simulink model "afe_inv_psm_param"  (R2026b)
settings: Solver=ode23t  StopTime=param.sim.simlength  FixedStep=tc  MaxStep=param.glb_time.tc  RelTol=1e-4
values from neighbouring files (symbols this model uses):
  param = add_template_extras(param, options)    [init_model.m]
undefined symbols (not defined in the file or in its folder): magnitude, omega_m_bez
libraries: fl_lib x330, nesl_utility x174, igbt_simple_2th_lib x12, moving_average_filter x10, moving_average_filter_cc x8, sl_discontinuities x3, single_phase_transformer_lib x3, linear_double_integrator_observer_ccaller x2, discrete_time_low_pass_filter x2, threephase_inductor_lib x2, three_phase_pwm_modulator x2, three_phase_inverter_ideal_switch_based_model x2
(part 13 of 13)

== system afe_inv_psm_param/afe_abc_inv_psm_mod1/INV_control/inverter_control/current_ctrl/current_ctrl/dq_pi_with_vector_antiwindup mod1/dq_vector_pi/vector lenght ==
  md : Inport
  mq : Inport  Port=2
  Math Function : Math  Operator=magnitude^2  SignedPower=on
  Math Function1 : Math  Operator=magnitude^2  SignedPower=on
  Math Function2 : Math  Operator=reciprocal  SignedPower=on
  Sqrt : Sqrt
  Sum5 : Sum  SaturateOnIntegerOverflow=on
  m_1 : Outport  VectorParamsAs1DForOutWhenUnconnected=off
  m : Outport  Port=2  VectorParamsAs1DForOutWhenUnconnected=off
  wires:
  Sqrt/1 -> m/1, Math Function2/1
  mq/1 -> Math Function1/1
  Math Function1/1 -> Sum5/2
  Math Function/1 -> Sum5/1
  Sum5/1 -> Sqrt/1
  Math Function2/1 -> m_1/1
  md/1 -> Math Function/1

== system afe_inv_psm_param/afe_abc_inv_psm_mod1/INV_control/inverter_control/current_ctrl/current_ctrl/dq_pi_with_vector_antiwindup mod1/dq_vector_pi_ccaller/Reset ==
  Step : Step  Time=0.05  InitialValue=1  FinalValue=0
  en : Outport
  wires:
  Step/1 -> en/1

== system afe_inv_psm_param/afe_abc_inv_psm_mod1/INV_control/inverter_control/current_ctrl/bemf_observer/EKF_bemf_observer/extended_kalman_observer/correlation_matrix/A_ekf ==
  Gain1 : Gain  Gain=param.psm.ctrl.ekf.A6_tilde_ekf
  Gain{7..10,13,20} (6 alike) : Gain  Gain=param.psm.machine.omega_bez
  Gain{2,4,6,11,16,18} (6 alike) : Gain  Gain=param.glb_time.ts_inv
  Gain15 : Gain  Gain=param.psm.ctrl.ekf.A2_tilde_ekf
  Gain17 : Gain  Gain=param.psm.ctrl.ekf.A3_tilde_ekf
  Gain3 : Gain  Gain=param.psm.ctrl.ekf.A4_tilde_ekf
  Gain5 : Gain  Gain=param.psm.ctrl.ekf.A5_tilde_ekf
  I1 : Constant  Value=eye(6)
  I2 : Constant  Value=param.psm.ctrl.ekf.A1_tilde_ekf
  Sum7 : Sum  Inputs=+++++++
  out : Outport
  wires:
  Sum7/1 -> out/1
  I2/1 -> Gain11/1
  I1/1 -> Sum7/1
  Gain1/1 -> Gain2/1
  Gain3/1 -> Gain4/1
  Gain5/1 -> Gain6/1
  [omega_hat_kalman] -> Gain1/1
  [psi_alpha_hat] -> Gain3/1
  [psi_beta_hat] -> Gain5/1
  Gain11/1 -> Gain7/1
  Gain2/1 -> Gain8/1
  Gain4/1 -> Gain9/1
  Gain6/1 -> Gain10/1
  Gain7/1 -> Sum7/2
  Gain9/1 -> Sum7/5
  Gain10/1 -> Sum7/6
  Gain8/1 -> Sum7/7
  Gain18/1 -> Gain13/1
  Gain16/1 -> Gain20/1
  Gain17/1 -> Gain18/1
  Gain15/1 -> Gain16/1
  Gain13/1 -> Sum7/4
  Gain20/1 -> Sum7/3
  [i_beta_hat] -> Gain17/1
  [i_alpha_hat] -> Gain15/1

== matlab function afe_inv_psm_param/afe_abc_inv_psm_mod1/AFE_control/afe_control/current_ctrl/current_transformation/alphabeta2xieta ==
  data: alpha input; xi output; beta input; gamma input; eta output
function [xi,eta] = alphabeta2xieta(alpha,beta,gamma)

    xi  =  alpha*cos(gamma) + beta*sin(gamma);
    eta = -alpha*sin(gamma) + beta*cos(gamma);

end

== matlab function afe_inv_psm_param/afe_abc_inv_psm_mod1/AFE_control/afe_control/grid_voltage_phase_lock_loops/FHT-PLL/pll_stageB/bounder1 ==
  data: u input; y output
function y = bounder(u)
    y = -pi + mod(u+3*pi,2*pi);
end

== matlab function afe_inv_psm_param/afe_abc_inv_psm_mod1/INV_control/inverter_control/current_ctrl/current_transformation/uvw2alphabeta ==
  data: u input; alpha output; v input; w input; beta output
function [alpha,beta] = uvw2alphabeta(u,v,w)

alpha = 2/3*(u - 1/2*v - 1/2*w);
beta  = 2/3*(sqrt(3)/2*(v - w));

end

== matlab function afe_inv_psm_param/afe_abc_inv_psm_mod1/INV_control/inverter_control/current_ctrl/current_ctrl/output voltage transformation/dq2alphabeta ==
  data: d input; alpha output; q input; gamma input; beta output
function [alpha,beta] = dq2alphabeta(d,q,gamma)

    alpha  =  d*cos(gamma) - q*sin(gamma);
    beta = d*sin(gamma) + q*cos(gamma);

end

== matlab function afe_inv_psm_param/afe_abc_inv_psm_mod1/AFE_control/afe_control/FRT-VDE4110/FRT-Detection/LVRT_detector ==
  data: vxi_p input; vxi_n input; veta_n input; vxi_p_dot input; vxi_n_dot input; enable input; red_dyn_enabled input; pwr_lim_enable output; frt_exceeded output; reset input; frt_active output; frt_state output; red_dyn_active output
function [pwr_lim_enable, frt_exceeded, frt_active, frt_state, red_dyn_active]  = lvrt_detector(vxi_p,vxi_n,veta_n,vxi_p_dot,vxi_n_dot, enable, red_dyn_enabled, reset)

    persistent state count count2 state_pwr_lim
    
    LVRT_IDLE = 0;
    LVRT_ACTIVE = 1;
    LVRT_EXCEEDED = 2;
    
    PWR_LIM_DISABLED = 0;
    PWR_LIM_ENABLED  = 1;
    
    LVRT_VPOS_TH_LOW			= 0.85;
    LVRT_VPOS_TH_HIGH			= 1.15;
    LVRT_SEQ_DETECTION_HYST		= 0.1;
    LVRT_VNEG_TH				= 0.1;
    LVRT_VPOS_DOT_TH			= 2.0;
    LVRT_VNEG_DOT_TH			= 2.0;
    LVRT_VPOS_PWRLIM_TH			= 0.8;
    LVRT_VNEG_PWRLIM_TH			= 0.1;
    LVRT_PWRLIM_HYST			= 0.1;
    LVRT_VPOS_RED_DYN_TH        = 0.7;
    LVRT_VNEG_RED_DYN_TH        = 0.2;
    LVRT_TIME_HOLD_MAX          = 61000;
    
    RED_DYN_NOT_ACTIVE = 0;
    RED_DYN_ACTIVE     = 1;
        
    if isempty(state)
        state = LVRT_IDLE;
        state_pwr_lim = PWR_LIM_DISABLED;
        count = 0;
        count2 = 0;
    end

    vn = sqrt(vxi_n^2+veta_n^2);

    if enable == 1
        
        switch state
            
            case LVRT_IDLE
                if ((vxi_p > LVRT_VPOS_TH_HIGH || vxi_p < LVRT_VPOS_TH_LOW || vn > LVRT_VNEG_TH) ...
                     && (vxi_p_dot > LVRT_VPOS_DOT_TH || vxi_n_dot > LVRT_VNEG_DOT_TH) && ...
                     count2 > 1000)
                    state = LVRT_ACTIVE;
                end
                frt_active = 0;
                frt_exceeded = 0;
                count = 0;
                frt_state = LVRT_IDLE;
                state_pwr_lim = PWR_LIM_DISABLED;                  
                red_dyn_active = RED_DYN_NOT_ACTIVE;
                count2 = count2 + 1;

            case LVRT_ACTIVE
                count2 = 0;
                % LVRT condition not active anymore
                if (vxi_p >= LVRT_VPOS_TH_LOW  + LVRT_SEQ_DETECTION_HYST && ...
                    vxi_p <  LVRT_VPOS_TH_HIGH - LVRT_SEQ_DETECTION_HYST)
                    state = LVRT_IDLE;
                % LVRT exceeded
                elseif (count >= LVRT_TIME_HOLD_MAX)
                    state = LVRT_EXCEEDED;
                end
                
                % handle power limitation
                if (vxi_p < LVRT_VPOS_PWRLIM_TH || vn > LVRT_VNEG_PWRLIM_TH) 
                    state_pwr_lim = PWR_LIM_ENABLED;
                elseif (vxi_p > LVRT_VPOS_PWRLIM_TH + LVRT_PWRLIM_HYST && vn < LVRT_VPOS_PWRLIM_TH - LVRT_PWRLIM_HYST)
                    state_pwr_lim = PWR_LIM_DISABLED;                  
                end
                
                % handle reduced dynamic grid support
                if red_dyn_enabled && (vxi_p < LVRT_VPOS_RED_DYN_TH || vn > LVRT_VNEG_RED_DYN_TH)
                    red_dyn_active = RED_DYN_ACTIVE;
                else
                    red_dyn_active = RED_DYN_NOT_ACTIVE;
                end
                 
                frt_active = 1;
                frt_exceeded = 0;
                frt_state = LVRT_ACTIVE;
                
                count = count + 1;
            
            case LVRT_EXCEEDED

                if ((reset == 1) || (enable == 0))
                    state = LVRT_IDLE;
                else
                    state = LVRT_EXCEEDED;
                end
                
                frt_exceeded = 1;
                frt_active = 0; 
                frt_state = LVRT_EXCEEDED;
                red_dyn_active = RED_DYN_NOT_ACTIVE;
            
            otherwise
                state = LVRT_IDLE;
                frt_active = 0;
                frt_exceeded = 0;
                frt_state = LVRT_IDLE;
                red_dyn_active = RED_DYN_NOT_ACTIVE;
        end
        
        if state_pwr_lim == PWR_LIM_ENABLED
            pwr_lim_enable = 1;
        else
            pwr_lim_enable = 0;
        end      
    else
        state = LVRT_IDLE;
        frt_active = 0;
        pwr_lim_enable = 0;
        frt_exceeded = 0;
        frt_state = LVRT_IDLE;
        red_dyn_active = RED_DYN_NOT_ACTIVE;
    end
end

== matlab function afe_inv_psm_param/afe_abc_inv_psm_mod1/brake/MATLAB Function ==
  data: u input; y output; udc_ref input
function y = fcn(u,udc_ref)

persistent enable_brake

udc_brake_min = 1.15;
udc_brake_max = 1.175;

if isempty(enable_brake)
    enable_brake = 0
end

if u >= udc_ref*udc_brake_max
    y = 15;
    enable_brake = 1;
elseif (u < udc_ref*udc_brake_max && u >= udc_ref*udc_brake_min && enable_brake == 1)
    y = 15;
    enable_brake = 1;
elseif (u < udc_ref*udc_brake_max && u >= udc_ref*udc_brake_min && enable_brake == 0)
    y = 0;
    enable_brake = 0;
else
    y = 0;
    enable_brake = 0;
end

% function y = fcn(u,udc_ref)
% 
% persistent enable_brake
% 
% udc_brake_min = 1.145;
% udc_brake_max = 1.165;
% 
% if isempty(enable_brake)
%     enable_brake = 0
% end
% 
% if u >= udc_ref*udc_brake_max
%     y = 15;
%     enable_brake = 1;
% elseif (u < udc_ref*udc_brake_max && u >= udc_ref*udc_brake_min && enable_brake == 1)
%     y = 15;
%     enable_brake = 1;
% elseif (u < udc_ref*udc_brake_max && u >= udc_ref*udc_brake_min && enable_brake == 0)
%     y = 0;
%     enable_brake = 0;
% else
%     y = 0;
%     enable_brake = 0;
end

== matlab function afe_inv_psm_param/afe_abc_inv_psm_mod1/AFE_control/afe_control/grid_voltage_phase_lock_loops/FHT-PLL/pll_stageB/double_integrator_observer/bounder1 ==
  data: u input; y output
function y = bounder(u)
    
    y = -pi + mod(u+3*pi,2*pi);
    
end

== matlab function afe_inv_psm_param/afe_abc_inv_psm_mod1/AFE_control/afe_control/grid_voltage_phase_lock_loops/FHT-PLL/pll_stageB/double_integrator_observer/bounder2 ==
  data: u input; y output
function y = bounder(u)
    
    y = -pi + mod(u+3*pi,2*pi);
    
end

== matlab function afe_inv_psm_param/afe_abc_inv_psm_mod1/INV_control/inverter_control/current_ctrl/bemf_observer/EKF_bemf_observer/extended_kalman_observer/double_integrator_observer/bounder2 ==
  data: u input; y output
function y = bounder(u)
    y = -pi + mod(u+3*pi,2*pi);
end

== matlab function afe_inv_psm_param/afe_abc_inv_psm_mod1/AFE_control/afe_control/grid_voltage_phase_lock_loops/FHT-PLL_simulink/pll_stageA/filter_and_transformation/abc2alphabeta ==
  data: a input; alpha output; b input; c input; beta output
function [alpha,beta] = abc2alphabeta(a,b,c)

alpha = 2/3*(a - 1/2*b - 1/2*c);
beta  = 1/sqrt(3)*(b - c);

end

== matlab function afe_inv_psm_param/afe_abc_inv_psm_mod1/AFE_control/afe_control/grid_voltage_phase_lock_loops/FHT-PLL_simulink/pll_stageA/sequences/alphabeta2xieta ==
  data: alpha input; xi output; beta input; gamma input; eta output
function [xi,eta] = alphabeta2xieta_pos(alpha,beta,gamma)

    xi  =  (alpha*cos(gamma) + beta*sin(gamma));
    eta = (-alpha*sin(gamma) + beta*cos(gamma));

end

== matlab function afe_inv_psm_param/afe_abc_inv_psm_mod1/AFE_control/afe_control/grid_voltage_phase_lock_loops/FHT-PLL_simulink/pll_stageB/bounder1 ==
  data: u input; y output
function y = bounder(u)
    y = -pi + mod(u+3*pi,2*pi);
end

== matlab function afe_inv_psm_param/afe_abc_inv_psm_mod1/AFE_control/afe_control/grid_voltage_phase_lock_loops/FHT-PLL_simulink/pll_stageB/double_integrator_observer/bounder1 ==
  data: u input; y output
function y = bounder(u)
    
    y = -pi + mod(u+3*pi,2*pi);
    
end

== matlab function afe_inv_psm_param/afe_abc_inv_psm_mod1/AFE_control/afe_control/grid_voltage_phase_lock_loops/dq_pll/pll_stageA/mormalization_and_transformation/abc2alphabeta ==
  data: a input; alpha output; b input; c input; beta output
function [alpha,beta] = abc2alphabeta(a,b,c)

alpha = 2/3*(a - 1/2*b - 1/2*c);
beta  = 1/sqrt(3)*(b - c);

end

== matlab function afe_inv_psm_param/afe_abc_inv_psm_mod1/AFE_control/afe_control/grid_voltage_phase_lock_loops/dq_pll/pll_stageA/sequences/alphabeta2xieta/alphabeta2xieta_neg ==
  data: alpha input; xi output; beta input; gamma input; eta output
function [xi,eta] = alphabeta2xieta_neg(alpha,beta,gamma)

    xi  = alpha*cos(gamma) - beta*sin(gamma);
    eta = alpha*sin(gamma) + beta*cos(gamma);

end

== matlab function afe_inv_psm_param/afe_abc_inv_psm_mod1/AFE_control/afe_control/grid_voltage_phase_lock_loops/dq_pll/pll_stageA/sequences/alphabeta2xieta/alphabeta2xieta_pos ==
  data: alpha input; xi output; beta input; gamma input; eta output
function [xi,eta] = alphabeta2xieta_pos(alpha,beta,gamma)

    xi  =  alpha*cos(gamma) + beta*sin(gamma);
    eta = -alpha*sin(gamma) + beta*cos(gamma);

end

== matlab function afe_inv_psm_param/afe_abc_inv_psm_mod1/INV_control/inverter_control/current_ctrl/bemf_observer/bemf_observer/double_integrator_observer/bounder1 ==
  data: u input; y output
function y = bounder(u)
    
    y = -pi + mod(u+3*pi,2*pi);
end

== matlab function afe_inv_psm_param/afe_abc_inv_psm_mod1/INV_control/inverter_control/current_ctrl/bemf_observer/bemf_observer/double_integrator_observer/bounder2 ==
  data: u input; y output
function y = bounder(u)
    
    u = -pi + mod(u+3*pi,2*pi);
    
    y = u;
end

== matlab function afe_inv_psm_param/afe_abc_inv_psm_mod1/AFE_control/afe_control/FRT-VDE4110/FRT-PosNegReactiveCurrentReferences/avg_flt_500ms/avg_flt_1 ==
  data: x input; y1 output; w input; ts input; enable input
function y1  = avg_flt(x,w,ts, enable)

    persistent x_int x_int_1 y_N N

    N = (1/(w/(2*pi)))/ts+1;

    if isempty(x_int)
        x_int_1 = 0;
        y_N = zeros(1,N);
        y1 = 0;
    end


    if enable == 1
        x_int = x * ts * w + x_int_1;
        x_int_1 = x_int;
        y_N(1,1) = x_int;
        y1 = 1/(2*pi)*((y_N(1,1) - y_N(1,N)));
        for i = 1:(N-1)
            y_N(1,N+1-i) = y_N(1,N-i); 
        end
    else
        y1 = 1/(2*pi)*((y_N(1,1) - y_N(1,N)));
    end
end

== matlab function afe_inv_psm_param/afe_abc_inv_psm_mod1/AFE_control/afe_control/grid_voltage_phase_lock_loops/dq_pll/pll_stageB/double_integrator_observer/bounder1 ==
  data: u input; y output
function y = bounder(u)
    
    y = -pi + mod(u+3*pi,2*pi);
    
end

== matlab function afe_inv_psm_param/afe_abc_inv_psm_mod1/AFE_control/afe_control/islanding_mode_detector/MATLAB Function ==
  data: alpha input; xi output; beta input; gamma input; eta output
function [xi,eta] = alphabeta2pos(alpha,beta,gamma)

    xi  =  alpha*cos(gamma) + beta*sin(gamma);
    eta = -alpha*sin(gamma) + beta*cos(gamma);

end

== matlab function afe_inv_psm_param/afe_abc_inv_psm_mod1/AFE_control/afe_control/grid_voltage_phase_lock_loops/dq_pll/pll_stageB/double_integrator_observer/bounder2 ==
  data: u input; y output
function y = bounder(u)
    
    y = -pi + mod(u+3*pi,2*pi);
    
end

== matlab function afe_inv_psm_param/afe_abc_inv_psm_mod1/AFE_control/afe_control/islanding_mode_detector/bounder ==
  data: u input; y output
function y = bounder(u)
    
    u = -pi + mod(u+3*pi,2*pi);
    
    y = u;
end

== matlab function afe_inv_psm_param/grid/power meter iec mfunc/three_phase_power_meter_iec ==
  data: phase input; m output Bus: PowerMeterIecBus; u_abc input; i_abc input; omega input; ts input; enable_time input
function m = three_phase_power_meter_iec(phase, u_abc, i_abc, omega, ts, enable_time)
%#codegen
% THREE_PHASE_POWER_METER_IEC
% Equivalente in singolo blocco MATLAB Function del sottosistema Simulink
% "three_phase_power_meter_iec" (libreria power_meter_iec).
%
% INGRESSI
%   phase       : angolo del PLL [rad]      (scalare)
%   u_abc       : tensioni di fase [V]      (3x1)
%   i_abc       : correnti di linea [A]     (3x1)
%   omega       : pulsazione di rete [rad/s] (scalare)
%   ts          : passo di campionamento [s]  -> parametro di maschera
%   enable_time : istante di abilitazione [s] -> parametro di maschera
%
% USCITA
%   m : struct (bus) con i campi, nello stesso ordine del Bus Creator
%       originale: Q1p, Q1n, P1n, P1p, U1n, U1p,
%                  i_act_1n, i_react_1n, i_act_1p, i_react_1p
%
% CATENA DI ELABORAZIONE (identica all'originale)
%   1) proiezione di ogni fase su cos(phase) e sin(phase), guadagno 2
%   2) media mobile dinamica su finestra pari a mezzo periodo di rete
%      (Tw = pi/|omega|), con lunghezza frazionaria interpolata
%   3) componenti simmetriche di sequenza diretta e inversa (Fortescue)
%   4) potenze attiva e reattiva per sequenza, tensioni concatenate RMS,
%      correnti attiva e reattiva per sequenza
%
% NOTE
%   - Il blocco deve girare a passo fisso ts (gli Zero-Order Hold di
%     ingresso dell'originale sono impliciti nel sample time del blocco).
%   - ts ed enable_time possono essere dichiarati come dati di scope
%     "Parameter" nel Symbols pane del MATLAB Function block, cosi'
%     risolvono direttamente sui parametri di maschera e la firma
%     esterna resta a 4 ingressi come nel blocco originale.

% ------------------------------------------------------------------
% Costanti
% ------------------------------------------------------------------
% MAVGFLT_SIZE_MAX = 17500;   % lunghezza buffer circolare (come originale)
MAVGFLT_SIZE_MAX = 2048;   % lunghezza buffer ridotto
NCH              = 12;      % canali filtrati: 6 per u_abc, 6 per i_abc

% Ordine canali:
%   1..3  ua_cos ub_cos uc_cos      7..9   ia_cos ib_cos ic_cos
%   4..6  ua_sin ub_sin uc_sin     10..12  ia_sin ib_sin ic_sin

% ------------------------------------------------------------------
% Stato persistente
% ------------------------------------------------------------------
persistent buf cb_index sample_count sum_short sum_long prev_input ...
           k_step period_held

if isempty(buf)
    buf          = zeros(NCH, MAVGFLT_SIZE_MAX);
    cb_index     = ones(NCH, 1);
    sample_count = ones(NCH, 1);
    sum_short    = zeros(NCH, 1);
    sum_long     = zeros(NCH, 1);
    prev_input   = zeros(NCH, 1);
    k_step       = 0;
    period_held  = 0;          % uscita iniziale dell'Enabled Subsystem
end

% ------------------------------------------------------------------
% Abilitazione (equivalente al blocco Step con Time = enable_time)
% ------------------------------------------------------------------
t_now  = k_step * ts;
k_step = k_step + 1;
enable = (t_now >= enable_time);

% ------------------------------------------------------------------
% Finestra di media: Enabled Subsystem 2*pi/w, alimentato da 2*|omega|.
% Quando |omega| = 0 l'Enabled Subsystem mantiene l'ultimo valore.
% ------------------------------------------------------------------
w2 = 2 * abs(omega);
if w2 > 0
    period_held = 2*pi / w2;   % = pi/|omega|, mezzo periodo di rete
end
period = period_held;

% ------------------------------------------------------------------
% Proiezione sin/cos, guadagno 2
% ------------------------------------------------------------------
c = cos(phase);
s = sin(phase);

x = zeros(NCH, 1);
x(1)  = 2 * u_abc(1) * c;   x(2)  = 2 * u_abc(2) * c;   x(3)  = 2 * u_abc(3) * c;
x(4)  = 2 * u_abc(1) * s;   x(5)  = 2 * u_abc(2) * s;   x(6)  = 2 * u_abc(3) * s;
x(7)  = 2 * i_abc(1) * c;   x(8)  = 2 * i_abc(2) * c;   x(9)  = 2 * i_abc(3) * c;
x(10) = 2 * i_abc(1) * s;   x(11) = 2 * i_abc(2) * s;   x(12) = 2 * i_abc(3) * s;

% ------------------------------------------------------------------
% Banco di 12 filtri a media mobile dinamica (dmavgflt_process)
% ------------------------------------------------------------------
y = zeros(NCH, 1);

if enable && period > 0

    desired = period / ts;
    if desired > (MAVGFLT_SIZE_MAX - 1)
        desired = MAVGFLT_SIZE_MAX - 1;
    end

    n_samples = floor(desired + 1);          % campioni che coprono il periodo
    frac      = desired + 1 - n_samples;     % parte frazionaria
    if n_samples < 1
        n_samples = 1;
    end

    for ch = 1:NCH

        ci = cb_index(ch);
        sc = sample_count(ch);

        if n_samples > sc
            % finestra in crescita: aggiungi campioni
            sum_short(ch) = sum_short(ch) + prev_input(ch);
            sum_long(ch)  = sum_long(ch)  + x(ch);
            sc = sc + 1;

        elseif n_samples < sc
            % finestra in contrazione: rimuovi i due campioni piu' vecchi
            i1 = mod(ci - 1 - sc,       MAVGFLT_SIZE_MAX) + 1;
            i2 = mod(ci - 1 - (sc - 1), MAVGFLT_SIZE_MAX) + 1;
            old_sum = buf(ch, i1) + buf(ch, i2);

            sum_short(ch) = sum_short(ch) + prev_input(ch) - old_sum;
            sum_long(ch)  = sum_long(ch)  + x(ch)          - old_sum;
            sc = sc - 1;

        else
            % finestra costante
            i1     = mod(ci - 1 - sc, MAVGFLT_SIZE_MAX) + 1;
            oldest = buf(ch, i1);

            sum_short(ch) = sum_short(ch) + prev_input(ch) - oldest;
            sum_long(ch)  = sum_long(ch)  + x(ch)          - oldest;
        end

        % aggiornamento buffer circolare
        buf(ch, ci)      = x(ch);
        cb_index(ch)     = mod(ci, MAVGFLT_SIZE_MAX) + 1;
        prev_input(ch)   = x(ch);
        sample_count(ch) = sc;

        % uscita: interpolazione lineare fra finestra corta e lunga
        if sc > 1
            avg_short = sum_short(ch) / (sc - 1);
        else
            avg_short = 0;
        end
        avg_long = sum_long(ch) / sc;

        y(ch) = avg_short * (1 - frac) + avg_long * frac;
    end
end
% se enable = false oppure period <= 0: y resta 0 e lo stato non evolve
% (comportamento identico all'originale)

ua_cos = y(1);  ub_cos = y(2);  uc_cos = y(3);
ua_sin = y(4);  ub_sin = y(5);  uc_sin = y(6);
ia_cos = y(7);  ib_cos = y(8);  ic_cos = y(9);
ia_sin = y(10); ib_sin = y(11); ic_sin = y(12);

% ------------------------------------------------------------------
% Componenti simmetriche (fasori con convenzione U = u_cos - j*u_sin)
% ------------------------------------------------------------------
sq3 = sqrt(3);

u1p_cos = (2*ua_cos - ub_cos - uc_cos - sq3*(uc_sin - ub_sin)) / 6;
u1p_sin = (2*ua_sin - ub_sin - uc_sin - sq3*(ub_cos - uc_cos)) / 6;
u1n_cos = (2*ua_cos - ub_cos - uc_cos - sq3*(ub_sin - uc_sin)) / 6;
u1n_sin = (2*ua_sin - ub_sin - uc_sin - sq3*(uc_cos - ub_cos)) / 6;

i1p_cos = (2*ia_cos - ib_cos - ic_cos - sq3*(ic_sin - ib_sin)) / 6;
i1p_sin = (2*ia_sin - ib_sin - ic_sin - sq3*(ib_cos - ic_cos)) / 6;
i1n_cos = (2*ia_cos - ib_cos - ic_cos - sq3*(ib_sin - ic_sin)) / 6;
i1n_sin = (2*ia_sin - ib_sin - ic_sin - sq3*(ic_cos - ib_cos)) / 6;

% ------------------------------------------------------------------
% Potenze per sequenza
% ------------------------------------------------------------------
P1p = 1.5 * (u1p_cos*i1p_cos + u1p_sin*i1p_sin);
Q1p = 1.5 * (u1p_cos*i1p_sin - u1p_sin*i1p_cos);
P1n = 1.5 * (u1n_cos*i1n_cos + u1n_sin*i1n_sin);
Q1n = 1.5 * (u1n_cos*i1n_sin - u1n_sin*i1n_cos);

% ------------------------------------------------------------------
% Tensioni concatenate RMS per sequenza: sqrt(3/2)*ampiezza di fase
% ------------------------------------------------------------------
U1p = sqrt(1.5 * (u1p_cos^2 + u1p_sin^2));
U1n = sqrt(1.5 * (u1n_cos^2 + u1n_sin^2));

% ------------------------------------------------------------------
% Correnti attiva e reattiva per sequenza (RMS di linea)
% La protezione contro la divisione per zero non era presente nello
% schema originale (i blocchi Divide restituivano Inf/NaN a U = 0).
% Portare U_MIN a 0 per replicare esattamente il comportamento vecchio.
% ------------------------------------------------------------------
U_MIN = 1e-9;

if U1p > U_MIN
    i_act_1p   = P1p / (sq3 * U1p);
    i_react_1p = Q1p / (sq3 * U1p);
else
    i_act_1p   = 0;
    i_react_1p = 0;
end

if U1n > U_MIN
    i_act_1n   = P1n / (sq3 * U1n);
    i_react_1n = Q1n / (sq3 * U1n);
else
    i_act_1n   = 0;
    i_react_1n = 0;
end

% ------------------------------------------------------------------
% Bus di uscita (stesso ordine dei campi dell'originale)
% ------------------------------------------------------------------
m.Q1p        = Q1p;
m.Q1n        = Q1n;
m.P1n        = P1n;
m.P1p        = P1p;
m.U1n        = U1n;
m.U1p        = U1p;
m.i_act_1n   = i_act_1n;
m.i_react_1n = i_react_1n;
m.i_act_1p   = i_act_1p;
m.i_react_1p = i_react_1p;

end

== matlab function afe_inv_psm_param/afe_abc_inv_psm_mod1/AFE_control/afe_control/current_ctrl/inner_current_ctrl/zero_current_ctrl/antiwind_up/MATLAB Function1 ==
  data: da input; das output; db input; dc input; scaling input; dbs output; dcs output
function [das, dbs, dcs] = fcn(da,db,dc,scaling)

das = da/scaling;
dbs = db/scaling;
dcs = dc/scaling;

== matlab function afe_inv_psm_param/afe_abc_inv_psm_mod1/AFE_control/afe_control/FRT-VDE4110/FRT-PosNegReactiveCurrentReferences/avg_flt_500ms1/avg_flt_1 ==
  data: x input; y1 output; w input; ts input; enable input
function y1  = avg_flt(x,w,ts, enable)

    persistent x_int x_int_1 y_N N

    N = (1/(w/(2*pi)))/ts+1;

    if isempty(x_int)
        x_int_1 = 0;
        y_N = zeros(1,N);
        y1 = 0;
    end


    if enable == 1
        x_int = x * ts * w + x_int_1;
        x_int_1 = x_int;
        y_N(1,1) = x_int;
        y1 = 1/(2*pi)*((y_N(1,1) - y_N(1,N)));
        for i = 1:(N-1)
            y_N(1,N+1-i) = y_N(1,N-i); 
        end
    else
        y1 = 1/(2*pi)*((y_N(1,1) - y_N(1,N)));
    end
end

== matlab function afe_inv_psm_param/afe_abc_inv_psm_mod1/AFE_control/afe_control/FRT-VDE4110/FRT-PosNegReactiveCurrentReferences/avg_flt_500ms2/avg_flt_1 ==
  data: x input; y1 output; w input; ts input; enable input
function y1  = avg_flt(x,w,ts, enable)

    persistent x_int x_int_1 y_N N

    N = (1/(w/(2*pi)))/ts+1;

    if isempty(x_int)
        x_int_1 = 0;
        y_N = zeros(1,N);
        y1 = 0;
    end


    if enable == 1
        x_int = x * ts * w + x_int_1;
        x_int_1 = x_int;
        y_N(1,1) = x_int;
        y1 = 1/(2*pi)*((y_N(1,1) - y_N(1,N)));
        for i = 1:(N-1)
            y_N(1,N+1-i) = y_N(1,N-i); 
        end
    else
        y1 = 1/(2*pi)*((y_N(1,1) - y_N(1,N)));
    end
end

== matlab function afe_inv_psm_param/afe_abc_inv_psm_mod1/AFE_control/afe_control/FRT-VDE4110/FRT-PosNegReactiveCurrentReferences/avg_flt_500ms3/avg_flt_1 ==
  data: x input; y1 output; w input; ts input; enable input
function y1  = avg_flt(x,w,ts, enable)

    persistent x_int x_int_1 y_N N

    N = (1/(w/(2*pi)))/ts+1;

    if isempty(x_int)
        x_int_1 = 0;
        y_N = zeros(1,N);
        y1 = 0;
    end


    if enable == 1
        x_int = x * ts * w + x_int_1;
        x_int_1 = x_int;
        y_N(1,1) = x_int;
        y1 = 1/(2*pi)*((y_N(1,1) - y_N(1,N)));
        for i = 1:(N-1)
            y_N(1,N+1-i) = y_N(1,N-i); 
        end
    else
        y1 = 1/(2*pi)*((y_N(1,1) - y_N(1,N)));
    end
end

== matlab function afe_inv_psm_param/afe_abc_inv_psm_mod1/AFE_control/afe_control/grid_voltage_sequences/v_alphabeta2xieta/MATLAB Function ==
  data: alpha input; xi output; beta input; gamma input; eta output
function [xi,eta] = alphabeta2pos(alpha,beta,gamma)

    xi  =  alpha*cos(gamma) + beta*sin(gamma);
    eta = -alpha*sin(gamma) + beta*cos(gamma);

end

== matlab function afe_inv_psm_param/afe_abc_inv_psm_mod1/AFE_control/afe_control/grid_voltage_sequences/v_alphabeta2xieta/MATLAB Function1 ==
  data: alpha input; xi output; beta input; gamma input; eta output
function [xi,eta] = alphabeta2neg(alpha,beta,gamma)

    xi  = alpha*cos(gamma) - beta*sin(gamma);
    eta = alpha*sin(gamma) + beta*cos(gamma);

end

== matlab function afe_inv_psm_param/afe_abc_inv_psm_mod1/AFE_control/afe_control/grid_voltage_sequences/grid_voltage_sampling_and_alpha_beta_transformation/v_abc2alphabeta ==
  data: v_abc input; alpha output; beta output
function [alpha,beta] = abc2alphabeta(v_abc)

alpha = 2/3*(v_abc(1) - 1/2*v_abc(2) - 1/2*v_abc(3));
beta  = 1/sqrt(3)*(v_abc(2) - v_abc(3));

end

== matlab function afe_inv_psm_param/afe_abc_inv_psm_mod1/AFE_control/afe_control/grid_current_sequences_and_reactive_pwr_ctrl/i_alphabeta2xieta/MATLAB Function ==
  data: alpha input; xi output; beta input; gamma input; eta output
function [xi,eta] = alphabeta2pos(alpha,beta,gamma)

    xi  =  alpha*cos(gamma) + beta*sin(gamma);
    eta = -alpha*sin(gamma) + beta*cos(gamma);

end

== matlab function afe_inv_psm_param/afe_abc_inv_psm_mod1/AFE_control/afe_control/grid_current_sequences_and_reactive_pwr_ctrl/i_alphabeta2xieta/MATLAB Function1 ==
  data: alpha input; xi output; beta input; gamma input; eta output
function [xi,eta] = alphabeta2neg(alpha,beta,gamma)

    xi  = alpha*cos(gamma) - beta*sin(gamma);
    eta = alpha*sin(gamma) + beta*cos(gamma);

end

== matlab function afe_inv_psm_param/afe_abc_inv_psm_mod1/AFE_control/afe_control/grid_current_sequences_and_reactive_pwr_ctrl/grid_current_sampling_and_alpha_beta_transformation/i_abc2alphabeta ==
  data: i_abc input; alpha output; beta output
function [alpha,beta] = abc2alphabeta(i_abc)

alpha = 2/3*(i_abc(1) - 1/2*i_abc(2) - 1/2*i_abc(3));
beta  = 1/sqrt(3)*(i_abc(2) - i_abc(3));

end

== matlab function afe_inv_psm_param/afe_abc_inv_psm_mod1/AFE_control/afe_control/current_ctrl/xieta2abc_ref/MATLAB Function2 ==
  data: alpha input; a output; beta input; b output; c output
function [a,b,c] = alphabeta2abc(alpha,beta)

a = alpha;
b = -(1/2)*alpha + sqrt(3)/2*beta;
c = -(1/2)*alpha - sqrt(3)/2*beta;

end

== matlab function afe_inv_psm_param/afe_abc_inv_psm_mod1/AFE_control/afe_control/current_ctrl/xieta2abc_ref/Negative Sequence ==
  data: xi input; alpha output; eta input; phase input; beta output
function [alpha,beta] = neg2alphabeta(xi,eta,phase)

    alpha = xi*cos(phase)  + eta*sin(phase);
    beta  = -xi*sin(phase) + eta*cos(phase);

end

== matlab function afe_inv_psm_param/afe_abc_inv_psm_mod1/AFE_control/afe_control/current_ctrl/xieta2abc_ref/Positive Sequence ==
  data: xi input; alpha output; eta input; phase input; beta output
function [alpha,beta] = pos2alphabeta(xi,eta,phase)

    alpha = xi*cos(phase) - eta*sin(phase);
    beta  = xi*sin(phase) + eta*cos(phase);

end

== matlab function afe_inv_psm_param/afe_abc_inv_psm_mod1/AFE_control/afe_control/grid_voltage_phase_lock_loops/dq_pll/pll_stageB/bounder1 ==
  data: u input; y output
function y = bounder(u)
    y = -pi + mod(u+3*pi,2*pi);
end

== matlab function afe_inv_psm_param/afe_abc_inv_psm_mod1/INV_control/inverter_control/current_ctrl/bemf_observer/EKF_bemf_observer/extended_kalman_observer/double_integrator_observer/bounder1 ==
  data: u input; y output
function y = bounder(u)
    y = -pi + mod(u+3*pi,2*pi);
end

== matlab function afe_inv_psm_param/afe_abc_inv_psm_mod1/INV_control/inverter_control/encoder-sensorless-switch/MATLAB Function ==
  data: omega_ctrl output; phase_psm input; omega_obs input; phase_obs input; phase_ctrl output; omega_psm input; omega_th input
function [omega_ctrl, phase_ctrl] = switch_enc2obs(phase_psm, omega_obs, phase_obs, omega_psm, omega_th)

if abs(omega_psm) > omega_th
    omega_ctrl = omega_obs;
    phase_ctrl = phase_obs;
else
    omega_ctrl = omega_psm;
    phase_ctrl = phase_psm;
end

== matlab function afe_inv_psm_param/afe_abc_inv_psm_mod1/AFE_control/afe_control/grid_voltage_phase_lock_loops/FHT-PLL_simulink/pll_stageB/double_integrator_observer/bounder2 ==
  data: u input; y output
function y = bounder(u)
    
    y = -pi + mod(u+3*pi,2*pi);
    
end

== matlab function afe_inv_psm_param/afe_abc_inv_psm_mod1/INV_control/inverter_control/encoder-sensorless-switch/double_integrator_observer/bounder1 ==
  data: u input; y output
function y = bounder(u)
    y = -pi + mod(u+3*pi,2*pi);
end

== matlab function afe_inv_psm_param/afe_abc_inv_psm_mod1/INV_control/inverter_control/encoder-sensorless-switch/double_integrator_observer/bounder2 ==
  data: u input; y output
function y = bounder(u)
    y = -pi + mod(u+3*pi,2*pi);
end

== matlab function afe_inv_psm_param/afe_abc_inv_psm_mod1/AFE_control/afe_control/current_ctrl/inner_current_ctrl/zero_current_ctrl/antiwind_up/MATLAB Function2 ==
  data: a input; alpha output; b input; c input; beta output; gamma output
function [alpha,beta, gamma] = abc2alphabeta(a,b,c)

alpha = 2/3*(a - 1/2*b - 1/2*c);
beta  = 1/sqrt(3)*(b - c);
gamma = (a+b+c)/3;

end

== matlab function afe_inv_psm_param/afe_abc_inv_psm_mod1/AFE_control/afe_control/grid_voltage_phase_lock_loops/FHT-PLL/pll_stageA/filter_and_transformation/abc2alphabeta ==
  data: a input; alpha output; b input; c input; beta output
function [alpha,beta] = abc2alphabeta(a,b,c)

alpha = 2/3*(a - 1/2*b - 1/2*c);
beta  = 1/sqrt(3)*(b - c);

end

== matlab function afe_inv_psm_param/afe_abc_inv_psm_mod1/AFE_control/afe_control/grid_voltage_phase_lock_loops/FHT-PLL/pll_stageA/sequences/alphabeta2xieta ==
  data: alpha input; xi output; beta input; gamma input; eta output
function [xi,eta] = alphabeta2xieta_pos(alpha,beta,gamma)

    xi  =  (alpha*cos(gamma) + beta*sin(gamma));
    eta = (-alpha*sin(gamma) + beta*cos(gamma));

end

== matlab function afe_inv_psm_param/afe_abc_inv_psm_mod1/INV_control/inverter_control/current_ctrl/current_transformation/alphabeta2dq ==
  data: alpha input; d output; beta input; gamma input; q output
function [d,q] = alphabeta2dq(alpha,beta,gamma)

    d  =  alpha*cos(gamma) + beta*sin(gamma);
    q = -alpha*sin(gamma) + beta*cos(gamma);

end

== matlab function afe_inv_psm_param/afe_abc_inv_psm_mod1/AFE_control/afe_control/current_ctrl/current_transformation/uvw2alphabeta ==
  data: u input; alpha output; v input; w input; beta output
function [alpha,beta] = uvw2alphabeta(u,v,w)

alpha = 2/3*(u - 1/2*v - 1/2*w);
beta  = 2/3*(sqrt(3)/2*(v - w));

end
